simulink model "Sample_task"  (Simulink 8.1)
settings: Solver=ode4  SolverMode=SingleTasking  StartTime=0.0  StopTime=inf  FixedStep=0.0005  RelTol=1e-3
StartFcn:
  |  warndlg('Dexterit-E models cannot run under simulation. Please compile your model and run it from within Dexterit-E.');set_param(bdroot,'SimulationCommand','stop')
undefined symbols (not defined in the file or in its folder): slselsubs
libraries: simulink x4, General x3, KINARM_loads x2, KINARM_IO x1, KINARM_EP_loads x1, Video x1, xpclib x1
(part 2 of 3)

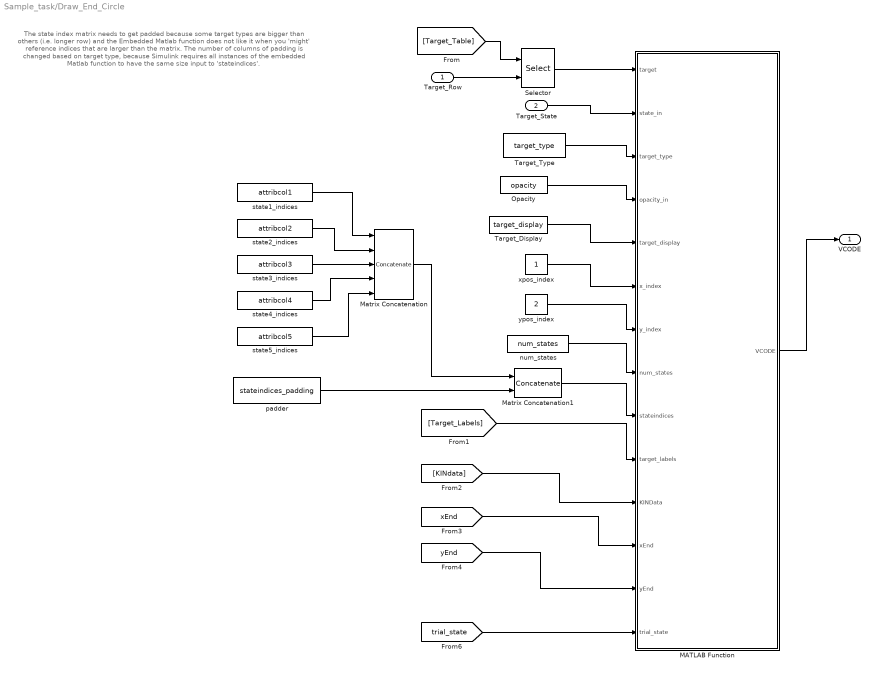
== system Sample_task/Draw_End_Circle ==
  note: The state index matrix needs to get padded because
      | some target types are bigger than others (i.e. longer row)
      | and the Embedded Matlab function does not like it when you
      |  'might' reference indices that are larger than the matrix.
      |
      | The number of columns of padding is changed based on target
      | type, because Simulink requires all instances of the embedded
      | Matlab function to have the same size input to 'stateindices'.
  Target_Row : Inport
  Target_State : Inport  Port=2
  MATLAB Function : MATLAB Function  TreatAsAtomicUnit=on
  Matrix Concatenation : Concatenate  NumInputs=5  Mode=Multidimensional array
  Matrix Concatenation1 : Concatenate  Mode=Multidimensional array  ConcatenateDimension=2
  Opacity : Constant  Value=opacity
  Selector : Selector  NumberOfDimensions=2  InputPortWidth=3  IndexOptions=Index vector (port),Select all  Indices=1,-1  OutputSizes=slselsubs([(-2),(-2)],1),slselsubs([(-2),(-2)],2)
  Target_Display : Constant  Value=target_display
  Target_Type : Constant  Value=target_type
  num_states : Constant  Value=num_states
  padder : Constant  Value=stateindices_padding
  state1_indices : Constant  Value=attribcol1  VectorParams1D=off
  state2_indices : Constant  Value=attribcol2  VectorParams1D=off
  state3_indices : Constant  Value=attribcol3  VectorParams1D=off
  state4_indices : Constant  Value=attribcol4  VectorParams1D=off
  state5_indices : Constant  Value=attribcol5  VectorParams1D=off
  xpos_index : Constant
  ypos_index : Constant  Value=2
  VCODE : Outport  PortDimensions=[1 70]
  wires:
  Target_Display/1 -> MATLAB Function/5(target_display)
  state2_indices/1 -> Matrix Concatenation/2
  state1_indices/1 -> Matrix Concatenation/1
  [Target_Labels] -> MATLAB Function/10(target_labels)
  Target_Row/1 -> Selector/2
  [Target_Table] -> Selector/1
  Selector/1 -> MATLAB Function/1(target)
  Target_State/1 -> MATLAB Function/2(state_in)
  MATLAB Function/1(VCODE) -> VCODE/1
  xpos_index/1 -> MATLAB Function/6(x_index)
  ypos_index/1 -> MATLAB Function/7(y_index)
  num_states/1 -> MATLAB Function/8(num_states)
  Matrix Concatenation/1 -> Matrix Concatenation1/1
  padder/1 -> Matrix Concatenation1/2
  Matrix Concatenation1/1 -> MATLAB Function/9(stateindices)
  state3_indices/1 -> Matrix Concatenation/3
  state4_indices/1 -> Matrix Concatenation/4
  state5_indices/1 -> Matrix Concatenation/5
  Opacity/1 -> MATLAB Function/4(opacity_in)
  Target_Type/1 -> MATLAB Function/3(target_type)
  [KINdata] -> MATLAB Function/11(KINData)
  [xEnd] -> MATLAB Function/12(xEnd)
  [yEnd] -> MATLAB Function/13(yEnd)
  [trial_state] -> MATLAB Function/14(trial_state)

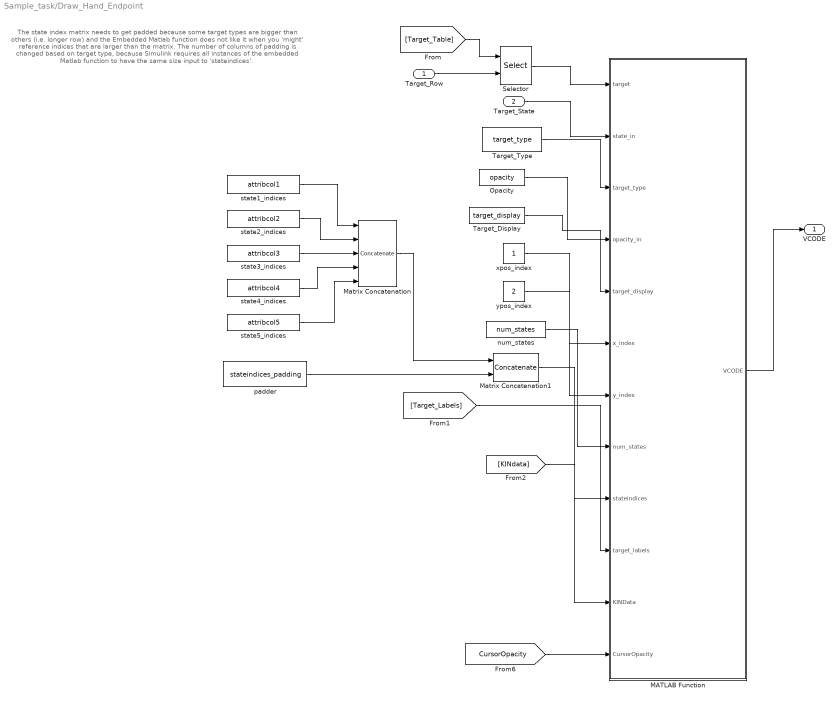
== system Sample_task/Draw_Hand_Endpoint ==
  note: The state index matrix needs to get padded because
      | some target types are bigger than others (i.e. longer row)
      | and the Embedded Matlab function does not like it when you
      |  'might' reference indices that are larger than the matrix.
      |
      | The number of columns of padding is changed based on target
      | type, because Simulink requires all instances of the embedded
      | Matlab function to have the same size input to 'stateindices'.
  Target_Row : Inport
  Target_State : Inport  Port=2
  MATLAB Function : MATLAB Function  TreatAsAtomicUnit=on
  Matrix Concatenation : Concatenate  NumInputs=5  Mode=Multidimensional array
  Matrix Concatenation1 : Concatenate  Mode=Multidimensional array  ConcatenateDimension=2
  Opacity : Constant  Value=opacity
  Selector : Selector  NumberOfDimensions=2  InputPortWidth=3  IndexOptions=Index vector (port),Select all  Indices=1,-1  OutputSizes=slselsubs([(-2),(-2)],1),slselsubs([(-2),(-2)],2)
  Target_Display : Constant  Value=target_display
  Target_Type : Constant  Value=target_type
  num_states : Constant  Value=num_states
  padder : Constant  Value=stateindices_padding
  state1_indices : Constant  Value=attribcol1  VectorParams1D=off
  state2_indices : Constant  Value=attribcol2  VectorParams1D=off
  state3_indices : Constant  Value=attribcol3  VectorParams1D=off
  state4_indices : Constant  Value=attribcol4  VectorParams1D=off
  state5_indices : Constant  Value=attribcol5  VectorParams1D=off
  xpos_index : Constant
  ypos_index : Constant  Value=2
  VCODE : Outport  PortDimensions=[1 70]
  wires:
  Target_Display/1 -> MATLAB Function/5(target_display)
  state2_indices/1 -> Matrix Concatenation/2
  state1_indices/1 -> Matrix Concatenation/1
  [Target_Labels] -> MATLAB Function/10(target_labels)
  Target_Row/1 -> Selector/2
  [Target_Table] -> Selector/1
  Selector/1 -> MATLAB Function/1(target)
  Target_State/1 -> MATLAB Function/2(state_in)
  MATLAB Function/1(VCODE) -> VCODE/1
  xpos_index/1 -> MATLAB Function/6(x_index)
  ypos_index/1 -> MATLAB Function/7(y_index)
  num_states/1 -> MATLAB Function/8(num_states)
  Matrix Concatenation/1 -> Matrix Concatenation1/1
  padder/1 -> Matrix Concatenation1/2
  Matrix Concatenation1/1 -> MATLAB Function/9(stateindices)
  state3_indices/1 -> Matrix Concatenation/3
  state4_indices/1 -> Matrix Concatenation/4
  state5_indices/1 -> Matrix Concatenation/5
  Opacity/1 -> MATLAB Function/4(opacity_in)
  Target_Type/1 -> MATLAB Function/3(target_type)
  [KINdata] -> MATLAB Function/11(KINData)
  [CursorOpacity] -> MATLAB Function/12(CursorOpacity)

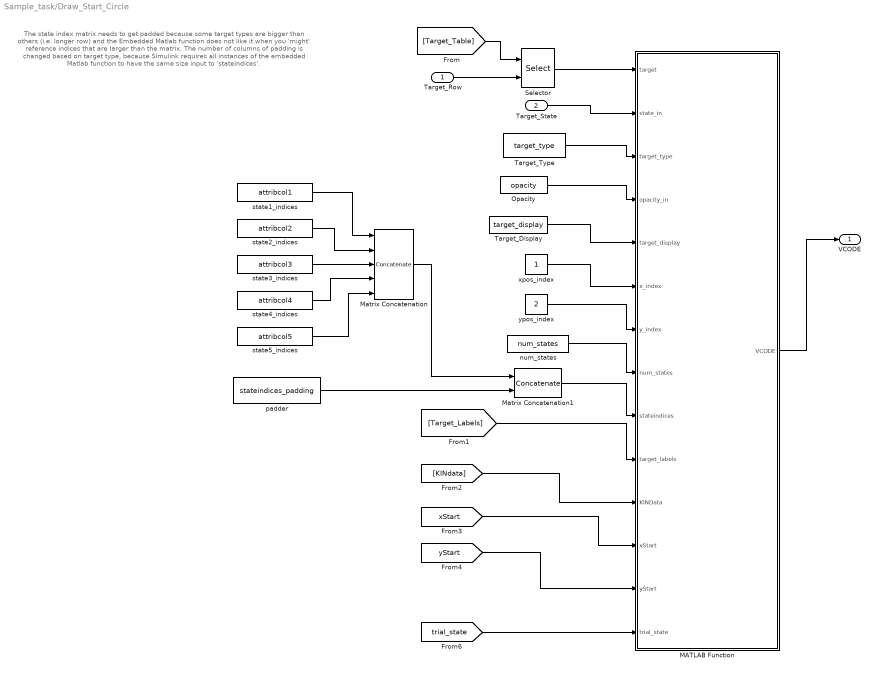
== system Sample_task/Draw_Start_Circle ==
  note: The state index matrix needs to get padded because
      | some target types are bigger than others (i.e. longer row)
      | and the Embedded Matlab function does not like it when you
      |  'might' reference indices that are larger than the matrix.
      |
      | The number of columns of padding is changed based on target
      | type, because Simulink requires all instances of the embedded
      | Matlab function to have the same size input to 'stateindices'.
  Target_Row : Inport
  Target_State : Inport  Port=2
  MATLAB Function : MATLAB Function  TreatAsAtomicUnit=on
  Matrix Concatenation : Concatenate  NumInputs=5  Mode=Multidimensional array
  Matrix Concatenation1 : Concatenate  Mode=Multidimensional array  ConcatenateDimension=2
  Opacity : Constant  Value=opacity
  Selector : Selector  NumberOfDimensions=2  InputPortWidth=3  IndexOptions=Index vector (port),Select all  Indices=1,-1  OutputSizes=slselsubs([(-2),(-2)],1),slselsubs([(-2),(-2)],2)
  Target_Display : Constant  Value=target_display
  Target_Type : Constant  Value=target_type
  num_states : Constant  Value=num_states
  padder : Constant  Value=stateindices_padding
  state1_indices : Constant  Value=attribcol1  VectorParams1D=off
  state2_indices : Constant  Value=attribcol2  VectorParams1D=off
  state3_indices : Constant  Value=attribcol3  VectorParams1D=off
  state4_indices : Constant  Value=attribcol4  VectorParams1D=off
  state5_indices : Constant  Value=attribcol5  VectorParams1D=off
  xpos_index : Constant
  ypos_index : Constant  Value=2
  VCODE : Outport  PortDimensions=[1 70]
  wires:
  Target_Display/1 -> MATLAB Function/5(target_display)
  state2_indices/1 -> Matrix Concatenation/2
  state1_indices/1 -> Matrix Concatenation/1
  [Target_Labels] -> MATLAB Function/10(target_labels)
  Target_Row/1 -> Selector/2
  [Target_Table] -> Selector/1
  Selector/1 -> MATLAB Function/1(target)
  Target_State/1 -> MATLAB Function/2(state_in)
  MATLAB Function/1(VCODE) -> VCODE/1
  xpos_index/1 -> MATLAB Function/6(x_index)
  ypos_index/1 -> MATLAB Function/7(y_index)
  num_states/1 -> MATLAB Function/8(num_states)
  Matrix Concatenation/1 -> Matrix Concatenation1/1
  padder/1 -> Matrix Concatenation1/2
  Matrix Concatenation1/1 -> MATLAB Function/9(stateindices)
  state3_indices/1 -> Matrix Concatenation/3
  state4_indices/1 -> Matrix Concatenation/4
  state5_indices/1 -> Matrix Concatenation/5
  Opacity/1 -> MATLAB Function/4(opacity_in)
  Target_Type/1 -> MATLAB Function/3(target_type)
  [KINdata] -> MATLAB Function/11(KINData)
  [xStart] -> MATLAB Function/12(xStart)
  [yStart] -> MATLAB Function/13(yStart)
  [trial_state] -> MATLAB Function/14(trial_state)

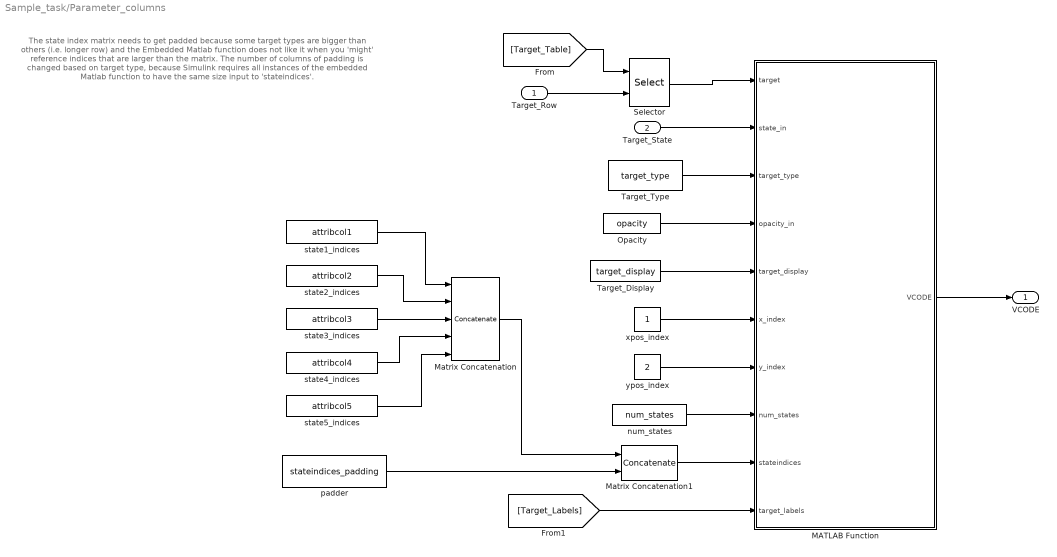
== system Sample_task/Parameter_columns ==
  note: The state index matrix needs to get padded because
      | some target types are bigger than others (i.e. longer row)
      | and the Embedded Matlab function does not like it when you
      |  'might' reference indices that are larger than the matrix.
      |
      | The number of columns of padding is changed based on target
      | type, because Simulink requires all instances of the embedded
      | Matlab function to have the same size input to 'stateindices'.
  Target_Row : Inport
  Target_State : Inport  Port=2
  MATLAB Function : MATLAB Function  TreatAsAtomicUnit=on
  Matrix Concatenation : Concatenate  NumInputs=5  Mode=Multidimensional array
  Matrix Concatenation1 : Concatenate  Mode=Multidimensional array  ConcatenateDimension=2
  Opacity : Constant  Value=opacity
  Selector : Selector  NumberOfDimensions=2  InputPortWidth=3  IndexOptions=Index vector (port),Select all  Indices=1,-1  OutputSizes=slselsubs([(-2),(-2)],1),slselsubs([(-2),(-2)],2)
  Target_Display : Constant  Value=target_display
  Target_Type : Constant  Value=target_type
  num_states : Constant  Value=num_states
  padder : Constant  Value=stateindices_padding
  state1_indices : Constant  Value=attribcol1  VectorParams1D=off
  state2_indices : Constant  Value=attribcol2  VectorParams1D=off
  state3_indices : Constant  Value=attribcol3  VectorParams1D=off
  state4_indices : Constant  Value=attribcol4  VectorParams1D=off
  state5_indices : Constant  Value=attribcol5  VectorParams1D=off
  xpos_index : Constant
  ypos_index : Constant  Value=2
  VCODE : Outport  PortDimensions=[1 70]
  wires:
  Target_Display/1 -> MATLAB Function/5(target_display)
  state2_indices/1 -> Matrix Concatenation/2
  state1_indices/1 -> Matrix Concatenation/1
  [Target_Labels] -> MATLAB Function/10(target_labels)
  Target_Row/1 -> Selector/2
  [Target_Table] -> Selector/1
  Selector/1 -> MATLAB Function/1(target)
  Target_State/1 -> MATLAB Function/2(state_in)
  MATLAB Function/1(VCODE) -> VCODE/1
  xpos_index/1 -> MATLAB Function/6(x_index)
  ypos_index/1 -> MATLAB Function/7(y_index)
  num_states/1 -> MATLAB Function/8(num_states)
  Matrix Concatenation/1 -> Matrix Concatenation1/1
  padder/1 -> Matrix Concatenation1/2
  Matrix Concatenation1/1 -> MATLAB Function/9(stateindices)
  state3_indices/1 -> Matrix Concatenation/3
  state4_indices/1 -> Matrix Concatenation/4
  state5_indices/1 -> Matrix Concatenation/5
  Opacity/1 -> MATLAB Function/4(opacity_in)
  Target_Type/1 -> MATLAB Function/3(target_type)

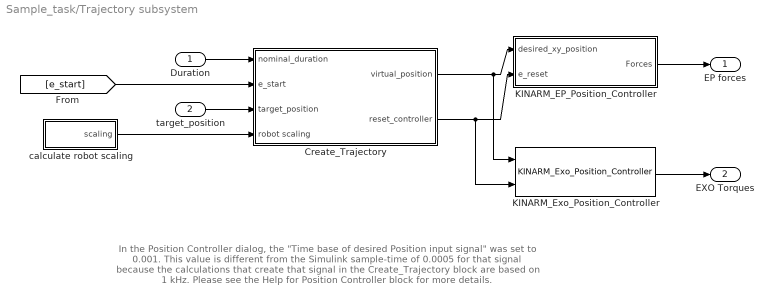
== system Sample_task/Trajectory subsystem ==
  note: In the Position Controller dialog, the "Time base of desired Position input signal" was set to 0.001.
      | This value is different from the Simulink sample-time of 0.0005 for that signal because the calculations
      | that create that signal in the Create_Trajectory block are based on 1 kHz. Please see the Help for
      | Position Controller block for more details.
  Duration : Inport
  target_position : Inport  Port=2
  Create_Trajectory : Subsystem
  KINARM_EP_Position_Controller : Subsystem  AncestorBlock=KINARM_EP_loads/KINARM_EP_Position_Controller  mask(KINARM_EP_Position_Controller){use_dom_hand=on, inertias_for_FF=KINARM End Point robot, gain_choice=Standard Movement, sample_time=0.001}
      mask prompts: use_dom_hand "Position control on dominant arm"; inertias_for_FF "Inertias to include for feed-forward control:"; gain_choice "Controller Performance"; sample_time "Time base of desired position input signal (-1 for inherited):"
      mask help:
      | <P>The KINARM_EP_Position_Controller block creates loads on the KINARM End-Point robot that implement position control of the hand using a feedforward model and feedback control.
      | <P>
      | The optional feedforward model uses estimates of KINARM End-Point robot inertia to create an estimate of required forces. A PD feedback controller is added to ensure optimal control.  The "Standard Movement" controller performance setting is optimized for reaching movements.  The "Step Response" setting is optimized for fast movements.
      | <P>
      | Desired position input is the (x, y) end-point position (i.e. handle).
      | <P>
      | <b>NOTE: it is critical to set the timebase of the desired position input signal correctly. Failure to do so will lead to robot instability, possibly damaging the KINARM robot and/or leading to subject injury.</b>
      mask init:
      | block_path = gcb;  % store block path, as gcb may change with block operations
      | 
      | %%% Handle background colours if link status changes.  
      | checkBackgroundColour(block_path, 'KINARM_EP_loads');
      | 
      | % Handle the inertias_for_FF setting: swap the 'inertia_option' inport with a constant block or 
      | % vice versa, if necessary, so that it matches the setting.
      | block_type = get_param([block_path '/inertia_option'], 'BlockType');
      | 
      | if (inertias_for_FF == 1) && ~strcmp(block_type, 'Inport') || ...  % if a change is required...
      |    (inertias_for_FF > 1) && strcmp(block_type, 'Inport')
      |     
      |     % ...delete the existing block, ...
      |     pos = get_param([block_path '/inertia_option'], 'Position');
      |     delete_line(block_path, 'inertia_option/1', 'FF_FB_Position_Controller/7');
      |     delete_block([block_path '/inertia_option']);
      |     
      |     % ...add an Inport or a 0-value Constant in place of the previous block (according to
      |     % the new setting), update the signal width flag, and then...
      |     if (inertias_for_FF == 1) && ~strcmp(block_type, 'Inport')
      |         add_block('built-in/Inport', [block_path '/inertia_option']);
      |      else
      |         add_block('built-in/Constant', [block_path '/inertia_option']);
      |         set_param([block_path '/inertia_option'], 'Value', 'inertias_for_FF - 2');
      |     end
      |     
      |     % ...connect the new block.
      |     set_param([block_path '/inertia_option'], 'Position', pos);
      |     add_line(block_path, 'inertia_option/1', 'FF_FB_Position_Controller/7');
      | end
      | 
      | 
      | 
      | % Set the sample rate of the desired_position input port based on the 
      | % sample rate from the mask
      | inports = find_system(block_path, 'LookUnderMasks', 'all', 'FollowLinks', 'on', 'SearchDepth', 1, 'BlockType', 'Inport');
      | set_param(inports{1}, 'SampleTime', get_param(gcb, 'sample_time') );
      | 
      | % Ensure the inports appear in a fixed order, and for each inport found add
      | % to the list of drawing commands a command to label it.
      | for i = 1:length(inports)
      |     inport_name = char(get_param(inports(i), 'Name'));
      |     
      |     if strcmp(inport_name, 'inertia_option')
      |         port = '3';
      | 	elseif strcmp(inport_name, 'desired_position')
      |         port = '1';
      |  	else
      | 		port = '2';
      | 		% do nothing
      | 	end
      |     
      |     set_param([block_path '/' inport_name], 'Port', port);
      | end
      mask Help:
      | Used to create loads for position control at the hand (i.e. finger-tip).
      | 
      | <H2>Library </H2>
      | KINARM_EP_loads (sub-library of Dexterit-E)
      | 
      | 
      | <H2>Description </H2>
      | The KINARM_EP_Position_Controller block creates loads on the KINARM End-Point robot that implement position control of the hand using a feedforward model and feedback control.
      | 
      | The optional feedforward model uses estimates of KINARM End-Point robot inertia to create an estimate of required forces. A PD feedback controller is added to ensure optimal control.  The "Standard Movement" controller performance setting is optimized for reaching movements.  The "Step Response" setting is optimized for fast movements.
      | <P>
      | <B>desired_xy_position: </B> this vector input is the desired position (i.e. attractor point) that the position controller acts on.  It should either be a [1x2] vector input or a VCODE.
      | The expected coordinate system and units for this input are the global coordinate system and meters.
      | <P>
      | <B>e_reset: </B> this scalar input resets the velocity and acceleration to zero for the feed-forward portion of the position controller model when e_reset transitions from 0 to 1.  This input should be used whenever the desired_xy_position input is being reset to a different position.
      | <P>
      | <B>inertia_option: </B> this optional scalar input defines which inertias to include for the feed-forward model.  Valid values are defined below.
      | <P>
      | <B>Forces: </B> this vector output is in a global Cartesian coordinate space as per all other KINARM End-Point load blocks.  It must be wired to the KINARM_EP_Apply_Loads block to actually apply the loads to the KINARM End-Point Robot.  This output may be added to other Force outputs from other KINARM End-Point load blocks to create a composite load.
      | <P>
      | 
      | <H2>Parameters and Dialog Box</H2>
      | <P>
      | <B>Position control on dominant arm:</B> indicates whether or not this position control is applied to the dominant arm (checked box) or non-dominant arm (unchecked box).
      | <P>
      | <B>Inertias to include for feed-forward control: </B> <BR>
      | Choices are: <BR>
      | (port)<BR>
      | 0 - None <BR>
      | 1 - KINARM End-Point robot  <BR>
      | <P>
      | If the (port) option is chosen, then an inport will be created allowing dynamic control of the inertia options.
      | The value wired to the inport will be mapped to the inertial choise using the values specified here (i.e. appropriate values are from 0-1).
      | Otherwise the option chosen will determine which inertias are included for the feed-forward control.
      | <P>
      | <B>Controller Performance: </B> <BR>
      | Choices are: <BR>
      | 1 - Standard Movement <BR>
      | 2 - Step Response  <BR>
      | <P>
      | The "Standard Movement" option is optimized for movements similar to normal reaching movements and provides high stiffness, but is underdamped.
      | There can be large overshoot following high accelerations/decellerations.
      | <P>
      | The "Step Response" option is optimized to minimize overshoot to less than ~10% for step responses, but at the cost of a reduction in controller stiffness.
      | <P>
      | NOTE: choice of Controller Performance option does not affect systems with secondary encoders - they are optimized for both conditions, providing higher stiffness and reasonable damping.
      | The controller for systems with secondary encoders provides less than ~10% overshoot for step responses.
      | <P>
      | 
      | <B>Time base of desired position input signal (-1 for inherited from sample time):</B> <BR>
      | Defines the time base used to calculate velocity and acceleration from the desired position input signal (-1 will inherit the time base from the sample time of the desired position input signal).
      | It is critical that this time base is set correctly.
      | The time base MUST be set to the time base used to create the desired input signal, WHICH MAY NOT BE THE SAME as the sample time of the desired input signal.
      | <B>Failure to set this time base correctly will lead to robot instability, possibly damaging the KINARM robot and/or leading to subject injury. </B>
      | <BR>
      | <I>Note: to determine the sample time of a signal, first update the model, then either select View --> Sample Time Legend or press Cntl + J.</I>
      | <P>
      | For example, a Stateflow chart that creates a desired position signal will, by default, use the model's sample time (e.g. 0.0005 s).
      | However, that Stateflow chart may use a time base that can be any multiple of the sample time (e.g. 0.001 s, 0.005 s, etc).
      | If a Stateflow chart was updating the desired position every 0.001 seconds, but the output sample time was 0.0005, then the position signal over time will look like:
      | <P>
      | [... x0, x0, x1, x1, x2, x2, x3, x3 ...].
      | <P>
      | A velocity calculated using 0.0005 time base will be:
      | <P>
      | [... 0, x1-x0, 0, x2-x1, 0, x3-x2, 0 ...] / 0.0005
      | <P>
      | (i.e. velocity will be 0 every other sample).
      | Whereas the true velocity in this example should be calculated using a 0.001 time base to create:
      | <P>
      |  [... x1-x0, x2-x1, x3-x2, ...] / 0.001.
      | 
      | <H2>Related Blocks </H2>
      | KINARM_EP_Apply_Loads, Virtual_Trajectory
      mask TypeOptions inertias_for_FF: (port) | None | KINARM End Point robot
      mask TypeOptions gain_choice: Standard Movement | Step Response
      mask Callback sample_time:
      | %ensure that sample time parameter is valid
      | sample_time_param = str2num( get_param(gcb, 'sample_time') );
      | model_step_size = str2num(get_param(bdroot, 'FixedStep'));
      | 
      | %default value:
      | sample_time = -1;
      | 
      | % if parameter value is numeric, sample_time_param will not be empty
      | if ~isempty(sample_time_param)
      | % 	round the sample time to an integer multiple of model step size, if possible
      | 	if ~isempty(model_step_size) && (model_step_size > 0)
      | 		sample_time = round( sample_time_param / model_step_size ) * model_step_size;
      | 	else
      | 		sample_time = sample_time_param;
      | 	end
      | 
      | 	% if input value is <=0, set it = -1 (inherited)
      | 	if (sample_time <= 0)
      | 		sample_time = -1;
      | 	end
      | end
      | 
      | set_param(gcb, 'sample_time', num2str(sample_time) );
  KINARM_Exo_Position_Controller : KINARM_loads/KINARM_Exo_Position_Controller  use_dom_hand=on  KINARM_Type=Human  inertias_for_FF=KINARM robot  angles_or_XY=End-point (global x/y)  sample_time=0.001
  calculate robot scaling : Subsystem
  EP forces : Outport
  EXO Torques : Outport  Port=2
  wires:
  Create_Trajectory/2(reset_controller) -> KINARM_EP_Position_Controller/2(e_reset), KINARM_Exo_Position_Controller/2
  Create_Trajectory/1(virtual_position) -> KINARM_EP_Position_Controller/1(desired_xy_position), KINARM_Exo_Position_Controller/1
  KINARM_EP_Position_Controller/1(Forces) -> EP forces/1
  KINARM_Exo_Position_Controller/1 -> EXO Torques/1
  target_position/1 -> Create_Trajectory/3(target_position)
  Duration/1 -> Create_Trajectory/1(nominal_duration)
  [e_start] -> Create_Trajectory/2(e_start)
  calculate robot scaling/1(scaling) -> Create_Trajectory/4(robot scaling)

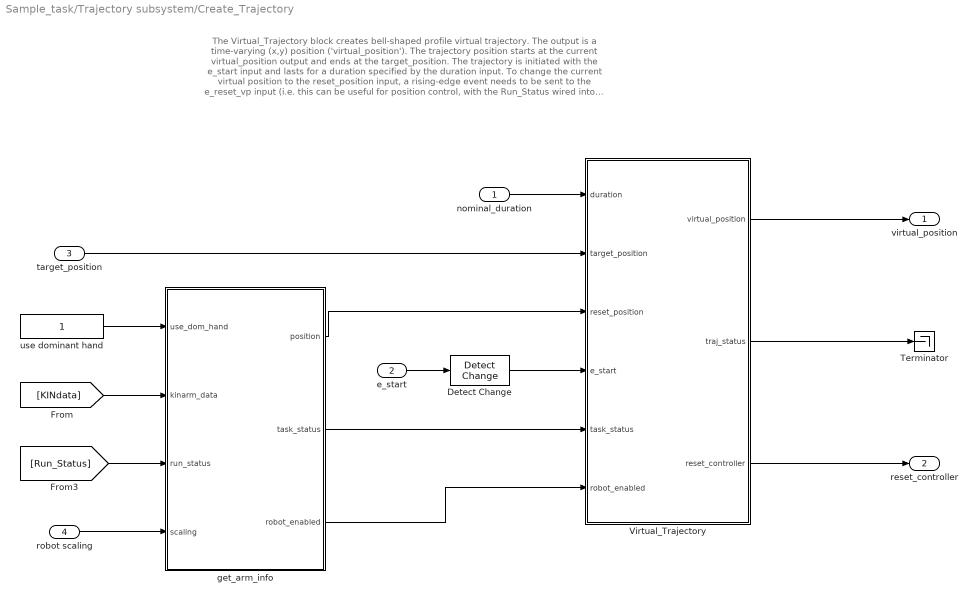
== system Sample_task/Trajectory subsystem/Create_Trajectory ==
  note: The Virtual_Trajectory block creates bell-shaped profile virtual trajectory.
      | The output is a time-varying (x,y) position ('virtual_position').
      |
      | The trajectory position starts at the current virtual_position output and ends at the target_position.
      | The trajectory is initiated with the e_start input and lasts for a duration specified by the duration input.
      |
      | To change the current virtual position to the reset_position input, a rising-edge event needs to be sent to the e_reset_vp input
      | (i.e. this can be useful for position control, with the Run_Status wired into the e_reset input).
      | If such an event occurs during a virtual trajectory, the trajectory is halted immediately.
  nominal_duration : Inport
  e_start : Inport  Port=2
  target_position : Inport  Port=3
  robot scaling : Inport  Port=4
  Detect Change : simulink/Logic and Bit Operations/Detect Change  vinit=0  InputProcessing=Inherited  OutDataTypeStr=uint8
  Terminator : Terminator
  Virtual_Trajectory : Subsystem
  get_arm_info : MATLAB Function  TreatAsAtomicUnit=on
  use dominant hand : Constant
  virtual_position : Outport
  reset_controller : Outport  Port=2
  wires:
  Virtual_Trajectory/1(virtual_position) -> virtual_position/1
  nominal_duration/1 -> Virtual_Trajectory/1(duration)
  e_start/1 -> Detect Change/1
  target_position/1 -> Virtual_Trajectory/2(target_position)
  Detect Change/1 -> Virtual_Trajectory/4(e_start)
  use dominant hand/1 -> get_arm_info/1(use_dom_hand)
  [KINdata] -> get_arm_info/2(kinarm_data)
  get_arm_info/1(position) -> Virtual_Trajectory/3(reset_position)
  Virtual_Trajectory/3(reset_controller) -> reset_controller/1
  get_arm_info/2(task_status) -> Virtual_Trajectory/5(task_status)
  get_arm_info/3(robot_enabled) -> Virtual_Trajectory/6(robot_enabled)
  [Run_Status] -> get_arm_info/3(run_status)
  Virtual_Trajectory/2(traj_status) -> Terminator/1
  robot scaling/1 -> get_arm_info/4(scaling)

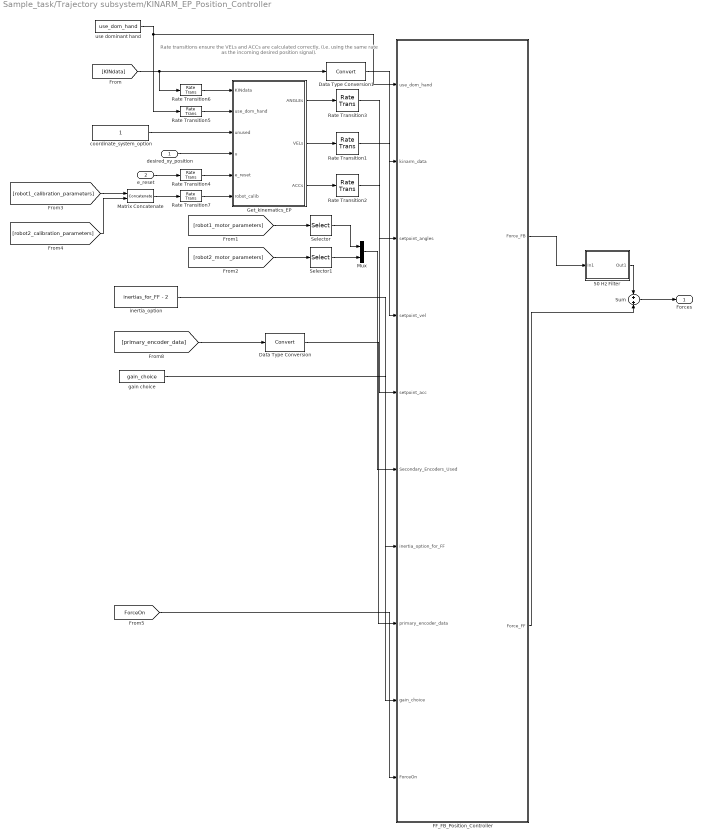
== system Sample_task/Trajectory subsystem/KINARM_EP_Position_Controller ==
  note: Rate transitions ensure the VELs and ACCs are calculated correctly,
      | (i.e. using the same rate as the incoming desired position signal).
  desired_xy_position : Inport  SampleTime=0.001
  e_reset : Inport  Port=2
  50 Hz Filter : Subsystem
  Data Type Conversion : DataTypeConversion
  Data Type Conversion1 : DataTypeConversion
  FF_FB_Position_Controller : MATLAB Function  TreatAsAtomicUnit=on
  Get_kinematics_EP : Subsystem  SystemSampleTime=.001
  Matrix Concatenate : Concatenate  Mode=Multidimensional array  ConcatenateDimension=2
  Mux : Mux  Inputs=2
  Rate Transition{1..7} (7 alike) : RateTransition
  Selector : Selector  IndexOptions=Index vector (dialog)  Indices=6  OutputSizes=[(-2)]
  Selector1 : Selector  IndexOptions=Index vector (dialog)  Indices=6  OutputSizes=[(-2)]
  Sum : Sum
  coordinate_system_option : Constant
  gain choice : Constant  Value=gain_choice
  inertia_option : Constant  Value=inertias_for_FF - 2
  use dominant hand : Constant  Value=use_dom_hand
  Forces : Outport  SampleTime=[0 1]
  wires:
  Data Type Conversion1/1 -> FF_FB_Position_Controller/2(kinarm_data)
  desired_xy_position/1 -> Get_kinematics_EP/4(u)
  use dominant hand/1 -> FF_FB_Position_Controller/1(use_dom_hand), Rate Transition5/1
  [KINdata] -> Data Type Conversion1/1, Rate Transition6/1
  Sum/1 -> Forces/1
  FF_FB_Position_Controller/1(Force_FB) -> 50 Hz Filter/1(In1)
  FF_FB_Position_Controller/2(Force_FF) -> Sum/2
  50 Hz Filter/1(Out1) -> Sum/1
  Get_kinematics_EP/1(ANGLEs) -> Rate Transition3/1
  Get_kinematics_EP/2(VELs) -> Rate Transition1/1
  Get_kinematics_EP/3(ACCs) -> Rate Transition2/1
  e_reset/1 -> Rate Transition4/1
  [robot1_motor_parameters] -> Selector/1
  [robot2_motor_parameters] -> Selector1/1
  Selector/1 -> Mux/1
  Selector1/1 -> Mux/2
  Mux/1 -> FF_FB_Position_Controller/6(Secondary_Encoders_Used)
  [primary_encoder_data] -> Data Type Conversion/1
  Data Type Conversion/1 -> FF_FB_Position_Controller/8(primary_encoder_data)
  gain choice/1 -> FF_FB_Position_Controller/9(gain_choice)
  Rate Transition1/1 -> FF_FB_Position_Controller/4(setpoint_vel)
  Rate Transition2/1 -> FF_FB_Position_Controller/5(setpoint_acc)
  Rate Transition3/1 -> FF_FB_Position_Controller/3(setpoint_angles)
  Rate Transition4/1 -> Get_kinematics_EP/5(e_reset)
  Rate Transition5/1 -> Get_kinematics_EP/2(use_dom_hand)
  Rate Transition6/1 -> Get_kinematics_EP/1(KINdata)
  coordinate_system_option/1 -> Get_kinematics_EP/3(unused)
  Rate Transition7/1 -> Get_kinematics_EP/6(robot_calib)
  Matrix Concatenate/1 -> Rate Transition7/1
  [robot1_calibration_parameters] -> Matrix Concatenate/1
  [robot2_calibration_parameters] -> Matrix Concatenate/2
  inertia_option/1 -> FF_FB_Position_Controller/7(inertia_option_for_FF)
  [ForceOn] -> FF_FB_Position_Controller/10(ForceOn)

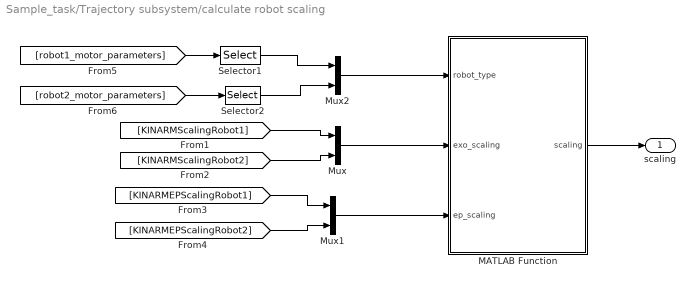
== system Sample_task/Trajectory subsystem/calculate robot scaling ==
  MATLAB Function : MATLAB Function  TreatAsAtomicUnit=on
  Mux : Mux  Inputs=2
  Mux1 : Mux  Inputs=2
  Mux2 : Mux  Inputs=2
  Selector1 : Selector  InputPortWidth=9  IndexOptions=Index vector (dialog)  Indices=[7]  OutputSizes=[(-2)]
  Selector2 : Selector  InputPortWidth=9  IndexOptions=Index vector (dialog)  Indices=[7]  OutputSizes=[(-2)]
  scaling : Outport
  wires:
  [KINARMScalingRobot1] -> Mux/1
  [KINARMScalingRobot2] -> Mux/2
  Mux/1 -> MATLAB Function/2(exo_scaling)
  Mux1/1 -> MATLAB Function/3(ep_scaling)
  Mux2/1 -> MATLAB Function/1(robot_type)
  MATLAB Function/1(scaling) -> scaling/1
  [robot2_motor_parameters] -> Selector2/1
  Selector2/1 -> Mux2/2
  [KINARMEPScalingRobot2] -> Mux1/2
  [KINARMEPScalingRobot1] -> Mux1/1
  Selector1/1 -> Mux2/1
  [robot1_motor_parameters] -> Selector1/1

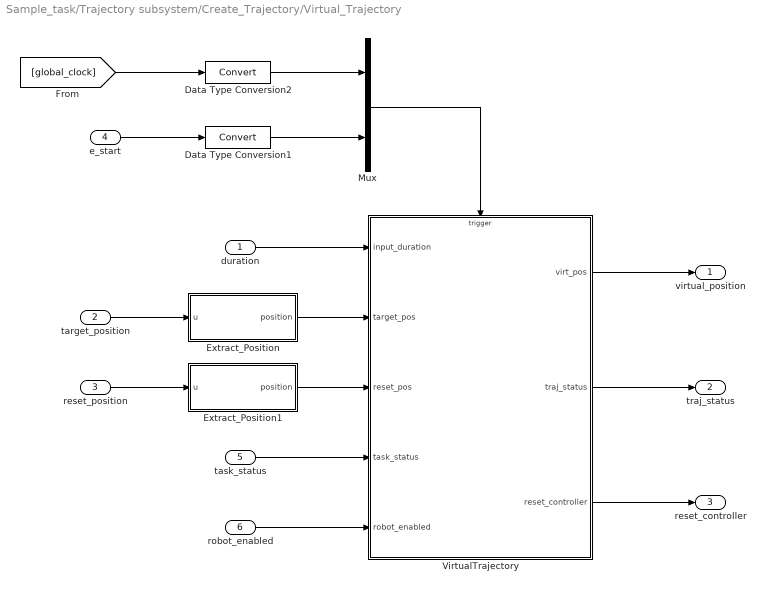
== system Sample_task/Trajectory subsystem/Create_Trajectory/Virtual_Trajectory ==
  duration : Inport
  target_position : Inport  Port=2
  reset_position : Inport  Port=3
  e_start : Inport  Port=4
  task_status : Inport  Port=5
  robot_enabled : Inport  Port=6
  Data Type Conversion1 : DataTypeConversion
  Data Type Conversion2 : DataTypeConversion
  Extract_Position : MATLAB Function  TreatAsAtomicUnit=on
  Extract_Position1 : MATLAB Function  TreatAsAtomicUnit=on
  Mux : Mux  Inputs=2
  VirtualTrajectory : Stateflow chart  TreatAsAtomicUnit=on
  virtual_position : Outport
  traj_status : Outport  Port=2
  reset_controller : Outport  Port=3
  wires:
  e_start/1 -> Data Type Conversion1/1
  target_position/1 -> Extract_Position/1(u)
  [global_clock] -> Data Type Conversion2/1
  Mux/1 -> VirtualTrajectory/Trigger
  duration/1 -> VirtualTrajectory/1(input_duration)
  VirtualTrajectory/1(virt_pos) -> virtual_position/1
  Extract_Position/1(position) -> VirtualTrajectory/2(target_pos)
  reset_position/1 -> Extract_Position1/1(u)
  Data Type Conversion2/1 -> Mux/1
  VirtualTrajectory/2(traj_status) -> traj_status/1
  robot_enabled/1 -> VirtualTrajectory/5(robot_enabled)
  task_status/1 -> VirtualTrajectory/4(task_status)
  Data Type Conversion1/1 -> Mux/2
  Extract_Position1/1(position) -> VirtualTrajectory/3(reset_pos)
  VirtualTrajectory/3(reset_controller) -> reset_controller/1

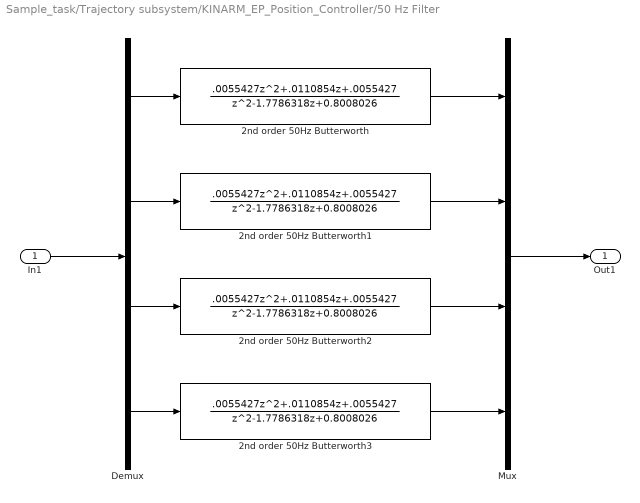
== system Sample_task/Trajectory subsystem/KINARM_EP_Position_Controller/50 Hz Filter ==
  In1 : Inport
  2nd order 50Hz Butterworth{,1..3} (4 alike) : DiscreteTransferFcn  Numerator=[.0055427 .0110854 .0055427]  Denominator=[1 -1.7786318 0.8008026]  SampleTime=.0005
  Demux : Demux
  Mux : Mux
  Out1 : Outport
  wires:
  Demux/2 -> 2nd order 50Hz Butterworth1/1
  In1/1 -> Demux/1
  Mux/1 -> Out1/1
  2nd order 50Hz Butterworth1/1 -> Mux/2
  Demux/1 -> 2nd order 50Hz Butterworth/1
  2nd order 50Hz Butterworth/1 -> Mux/1
  Demux/3 -> 2nd order 50Hz Butterworth2/1
  2nd order 50Hz Butterworth2/1 -> Mux/3
  Demux/4 -> 2nd order 50Hz Butterworth3/1
  2nd order 50Hz Butterworth3/1 -> Mux/4

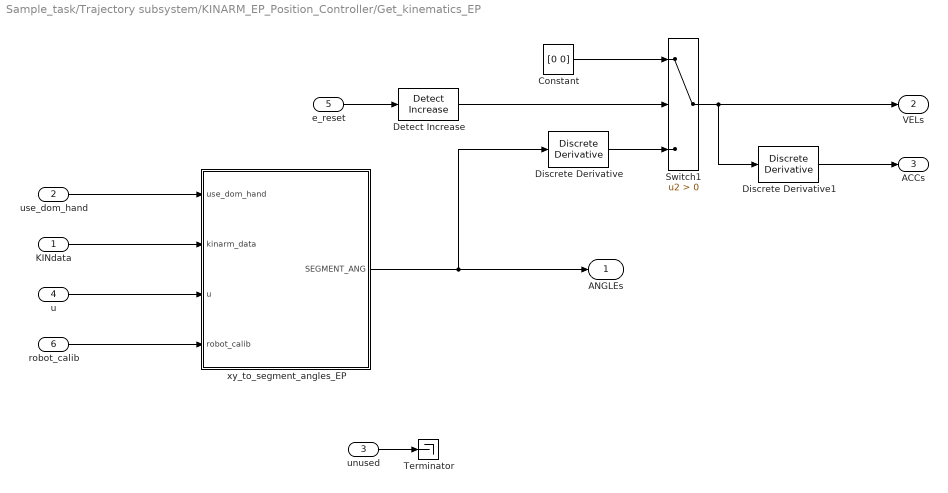
== system Sample_task/Trajectory subsystem/KINARM_EP_Position_Controller/Get_kinematics_EP ==
  KINdata : Inport
  use_dom_hand : Inport  Port=2
  unused : Inport  Port=3
  u : Inport  Port=4
  e_reset : Inport  Port=5
  robot_calib : Inport  Port=6
  Constant : Constant  Value=[0 0]
  Detect Increase : simulink/Logic and Bit Operations/Detect Increase  vinit=0.0  InputProcessing=Inherited  OutDataTypeStr=uint8
  Discrete Derivative : simulink/Discrete/Discrete Derivative  gainval=1.0  ICPrevScaledInput=0.0  InputProcessing=Inherited  OutMin=[]  OutMax=[]  OutDataType=sfix(16)  OutScaling=2^-10  DoSatur=off
  Discrete Derivative1 : simulink/Discrete/Discrete Derivative  gainval=1.0  ICPrevScaledInput=0.0  InputProcessing=Inherited  OutMin=[]  OutMax=[]  OutDataType=sfix(16)  OutScaling=2^-10  DoSatur=off
  Switch1 : Switch  Criteria=u2 > Threshold
  Terminator : Terminator
  xy_to_segment_angles_EP : MATLAB Function  TreatAsAtomicUnit=on
  ANGLEs : Outport
  VELs : Outport  Port=2
  ACCs : Outport  Port=3
  wires:
  xy_to_segment_angles_EP/1(SEGMENT_ANG) -> ANGLEs/1, Discrete Derivative/1
  Discrete Derivative/1 -> Switch1/3
  use_dom_hand/1 -> xy_to_segment_angles_EP/1(use_dom_hand)
  u/1 -> xy_to_segment_angles_EP/3(u)
  Switch1/1 -> Discrete Derivative1/1, VELs/1
  Constant/1 -> Switch1/1
  Detect Increase/1 -> Switch1/2
  Discrete Derivative1/1 -> ACCs/1
  KINdata/1 -> xy_to_segment_angles_EP/2(kinarm_data)
  e_reset/1 -> Detect Increase/1
  unused/1 -> Terminator/1
  robot_calib/1 -> xy_to_segment_angles_EP/4(robot_calib)

== stateflow chart Trial_Control ==
  settings: sampleTime=0.001
  state Main_Trial/
    state InCentre/
      rest = Trial_Protocol[REST_COL];
      % State - wait for subject
      trial_state = 0;
      % Initialize cursor
      EMG_trigger = 0;
    state EndOfTrial/
      logging_enable = 0;
      % State - rest
      trial_state = 2;
      EMG_trigger = 0;
    state DuringTrial/
      % Recording enabled
      logging_enable = 1;
      % Turn force on forever
      ForceOn = 1;
      % State - during trial
      trial_state = 1;
      % Trigger
      EMG_trigger = 5;
    state StayInCentre/
    StayInCentre -> InCentre [order 2] : [HandAtStart==0]
    InCentre -> StayInCentre : [HandAtStart==1]
    StayInCentre -> DuringTrial [order 1] : after(100,e_clk)
    DuringTrial -> EndOfTrial : after(Trial_Protocol[TRAJ_DURATION_COL]*1000,e_clk)
  state init/
    ForceOn = 0;
  state Inter_Trial_State/
    e_Trial_End
  state WaitForFlagToSet
  init -> InCentre
  (default) -> init
  Inter_Trial_State -> InCentre
  WaitForFlagToSet -> Inter_Trial_State : after(2, e_clk)
  Main_Trial -> WaitForFlagToSet : e_ExitTrialNow/
      | logging_enable = 0;
      | tickCount = 10;
  EndOfTrial -> Inter_Trial_State : after(rest*1000,e_clk)
  data: logging_enable output boolean; trial_state output double; tickCount local double; Trial_Protocol input double; HandAtStart input double; rest local double; ForceOn output double; EMG_trigger output double
  events: e_clk input RISING_EDGE_EVENT; e_ExitTrialNow input EITHER_EDGE_EVENT; e_Trial_End output EITHER_EDGE_EVENT

== matlab function Draw_End_Circle/MATLAB Function ==
  data: target input double; VCODE output double; state_in input double; target_type input double; opacity_in input double; target_display input double; x_index input double; y_index input double; num_states input double; stateindices input double; target_labels input double; KINData input double; xEnd input double; yEnd input double; trial_state input double
function VCODE = fcn(target, state_in, target_type, opacity_in, target_display, x_index, y_index, num_states, stateindices, target_labels, KINData, xEnd, yEnd, trial_state)

% stateindices should follow this order (depending on target-type):
% 1: fill colour
% 2: stroke colour
% 3: stroke width
% 4: major radius / radius / start point (line)
% 5: minor radius / end point (line)
% 6: orientation angle



% VCODEs are length 70. All units in a VCODE should be SI, e.g. (m) and (rad). Elements in a VCODE are defined as follows:
%
% For all target types:
%  1: target type
%       1 - circle
%       2 - ellipse
%       3 - rectangle
%       4 - line
%       5 - triangle
%       11 - circle with label
%       12 - ellipse with label
%       13 - rectangle with label
%       14 - line with label
%       15 - triangle with label
%  2: target on/off status and target display (which display target will appear on)
%		0 - off
%		1 - on, appearing on both subject and operator displays
%       2 - on, appearing on subject display only
%       3 - on, appearing on operator display only
%  3: x position (m)
%  4: y position (m)
%  5: fill colour (RRGGBB) or texture index
%  6: stroke colour (RRGGBB) or texture index
%  7: stroke width
%  8: reserved for target background ID
%  9: opacity
%
% For circles:
%  10: radius (m)
%
% For ellipses:
%  10: major radius (m)
%  11: minor radius (m)
%  12: orientation of major axis (rad)
%
% For rectangles:
%  10: length (m)
%  11: height (m)
%  12: orientation (rad) (relative to x, y already shown)
%
% For lines:
%  10: endpoint x-axis coordinate relative to start point (m)
%  11: endpoint y-axis coordinate relative to start point (m)
%
% For triangles:
%  10: length (m)
%  11: height (m)
%  12: offset of peak from midpoint of length (m)
%  13: orientation (rad)
%
% For all labelled target types:
%  14: reserved
%  15-64: label characters (indexes in ISO 8859-1 character set)
%  65: label colour (0xRRGGBB), opacity is set by the vcode's opacity (9).
%  66: label height (m)
%  67: reserved
%  68: reserved
%  69: reserved
%  70: reserved

num_targets = size(target, 1);

% NOTE: we assume that the STATE and/or OPACITY inputs are vectors. 

% If the length of the input STATE is not the same as the number of targets then make STATE a column vector of the same length as 
% the TARGET input, using the first STATE (i.e. all targets get the same state)
if num_targets == length(state_in)
	state = reshape(state_in, num_targets, 1);
else
	state = state_in(1) * ones(num_targets, 1);
end


% If the length of the input OPACITY is not the same as the number of targets then make OPACITY a column vector of the same length as
% the TARGET input, using the first OPACITY (i.e. all targets get the same opacity)
if num_targets == length(opacity_in)
	opacity = reshape(opacity_in, num_targets, 1);
else
	opacity = opacity_in(1) * ones(num_targets, 1);
end


% Clamping the opacity to [0, 100].
opacity = min(opacity, 100);
opacity = max(opacity, 0);

VCODE = zeros(num_targets, 70);

% Set the target type. Targets with labels have type codes 10 greater than their unlabelled counterparts.
VCODE(:, 1) = target_type + 10;

% Set the hand position.
VCODE(:, 3) = xEnd;  % x position (m)
VCODE(:, 4) = yEnd;  % y position (m)

for ii = 1:num_targets
	% Set the target on/off state. If the state input is 0, the target is off. Users of the VCODE should respect this
	% as an indication that the rest of the VCODE will be uninitialized.
	if (state(ii) <= 0) || (state(ii) > num_states)
		VCODE(ii, 2) = 0;  % target is off
	else
		VCODE(ii, 2) = target_display;  % Default is that target is on; target displays as specified by block mask
	end

	fill_colour_col = stateindices(state(ii), 1);
	stroke_colour_col = stateindices(state(ii), 2);
	stroke_width_col = stateindices(state(ii), 3);
	
	% Set the fill colour. Fill colour currently comes from the GUI in RRRGGGBBB format.
	%{
    if fill_colour_col == 0
		VCODE(ii, 5) = -2^31;
	elseif target(fill_colour_col) < 0
		VCODE(ii, 5) = target(ii, fill_colour_col);
	else
		VCODE(ii, 5) = colourshift(target(ii, fill_colour_col));
    end
    %}
    VCODE(ii,5) = colourshift(1000000000);
	
	% Set the stroke colour. Stroke colour currently comes from the GUI in RRRGGGBBB format.
    if trial_state==1
        if stroke_colour_col == 0
            VCODE(ii, 6) = -2^31;
        elseif target(stroke_colour_col) < 0
            VCODE(ii, 6) = target(ii, stroke_colour_col);
        else
            VCODE(ii, 6) = colourshift( target(ii, stroke_colour_col) );
        end
    else
        % CIRCLE APPEARS ONLY DURING TASK
        VCODE(ii, 6) = colourshift(1000000000);
    end

	% Set the stroke width. if target table index for stroke width is zero, then the stroke width is undefined
	if stroke_width_col == 0
		VCODE(ii, 7) = 0;                   % if stroke width column is 0, then stroke width is 0
	elseif stroke_width_col < 0
		VCODE(ii, 7) = 0.001;               % if stroke width column is -ve, then a 1mm default is chosen
	else
		VCODE(ii, 7) = target(ii, stroke_width_col) * 0.01;  % if stroke width column is +ve, convert width from (cm) in target table to (m)
    end

	% Set the opacity value
	VCODE(ii, 9) = opacity(ii);

	% Set attributes specific to each target type. In the process, note the first state vector column used for label information.
	label_index = 1;

	% Set attributes specific to each target type.
	if target_type == 1

		% Handle circle target:
		radius_col = stateindices(state(ii), 4);
		VCODE(ii, 10)=target(ii, radius_col);  % radius (in m)
	    label_index = 5;

	elseif target_type == 2 || target_type == 3

	    % Handle ellipse or rectangle target:
		major_col = stateindices(state(ii), 4);
		minor_col = stateindices(state(ii), 5);
		orientation_col = stateindices(state(ii), 6);
		
		VCODE(ii, 10) = target(ii, major_col) * 0.01;  % major radius (convert from (cm) in target table to (m))
		VCODE(ii, 11) = target(ii, minor_col) * 0.01;  % minor radius (convert from (cm) in target table to (m))
		if orientation_col == 0
			VCODE(ii, 12) = 0;  % if orientation column is 0, set orientation to 0 rad
		else
			VCODE(ii, 12) = mod(target(ii, orientation_col), 360) * pi / 180.0;  % orientation (convert from (degrees) in target table to (rad))
		end
	    label_index = 7;
	
	elseif target_type == 4

		% Handle line target:
		%xendpoint_col = stateindices(state(ii), 4);
		%yendpoint_col = stateindices(state(ii), 5);
		VCODE(ii, 10) = 0;  % line endpoint in x axis, relative to start (m)
		VCODE(ii, 11) = stateindices(state(ii), 1);  % line endpoint in y axis, relative to start (taken from Target Table)
	    label_index = 6;

	elseif target_type == 5

		% Handle triangle target:
		length_col = stateindices(state(ii), 4);
		height_col = stateindices(state(ii), 5);
		offset_col = stateindices(state(ii), 6);
		orientation_col = stateindices(state(ii), 7);

		VCODE(ii, 10) = target(ii, length_col) * 0.01;  % length (convert from (cm) in target table to (m))

		% If the height column is set to 0 then the triangle is automatically made equilateral, with the base length used as length
		% for all sides. If the height column is non-zero, separate values for height and peak offset are taken from the target table.
		if height_col == 0
			VCODE(ii, 11) = sin(pi / 3.0) * VCODE(ii, 10);  % height for equilateral triangle
			VCODE(ii, 12) = 0;                          % peak offset for equilateral triangle
		else
			VCODE(ii, 11) = target(ii, height_col) * 0.01;  % height (convert from (cm) in target table to (m))
			VCODE(ii, 12) = target(ii, offset_col) * 0.01;  % peak offset (convert from (cm) in target table to (m))
		end

		if orientation_col == 0
			VCODE(ii, 13) = 0;  % if orientation column is 0, set orientation to 0 rad
		else
			VCODE(ii, 13) = mod(target(ii, orientation_col), 360) * pi / 180.0;  % orientation (convert from (degrees) in target table to (rad))
		end
	    label_index = 8;
		
	end
	
	% Copy the label characters to the VCODE.
	for jj = 1:50
		VCODE(ii, jj + 14) = target_labels( target( ii, stateindices(state(ii), label_index) ), jj );
	end

	% Set the label colour. Like other colours, label colour comes from the GUI in RRRGGGBBB format and is converted to a 32-bit
	% 0xRRGGBB value here. If the target column table index for the colour is 0, the label is transparent.
	if stateindices(state(ii), label_index + 1) == 0
		VCODE(ii, 65) = -2^31;
	elseif target( ii, stateindices(state(ii), label_index + 1) ) < 0
		VCODE(ii, 65) = target( ii, stateindices(state(ii), label_index + 1) );
	else
		VCODE(ii, 65) = colourshift( target( ii, stateindices(state(ii), label_index + 1) ) );
	end

	% Set the label height. Label height is converted from (cm) in the target table to (m).
	VCODE(ii, 66) = target( ii, stateindices(state, label_index + 2) ) * 0.01;


	
end

% The colourshift function converts an "RRRGGGBBB" colour value to RRGBB (as an uint32).
function RRGGBBAA = colourshift(RRRGGGBBB)

%this is "no fill"
if RRRGGGBBB == 1000000000
    RRGGBBAA = cast(16777216, 'uint32'); %hex 0x1000000
    return; 
end

blue = cast(mod(RRRGGGBBB, 1000), 'uint32');
green = cast(mod(RRRGGGBBB - blue, 1000000) / 1000, 'uint32');
red = cast((RRRGGGBBB - (green * 1000) - blue) / 1000000, 'uint32');

RRGGBBAA = bitshift(red, 16) + bitshift(green, 8) + blue;

== matlab function Trajectory subsystem/Create_Trajectory/Virtual_Trajectory/Extract_Position ==
  settings: fimath=|
      | fimath(...
      | 'RoundMode', 'floor',...
      | 'OverflowMode', 'wrap',...
      | 'ProductMode', 'KeepLSB', 'ProductWordLength', 32,...
      | 'SumMode', 'KeepLSB', 'SumWordLength', 32,...
      | 'CastBeforeSum', false)
  data: u input double; position output double
function position = fcn(u)

position=[0,0];	%initialization
if length(u)==2	%input is assumed to be (x,y) position, global coordinates, (m)		
	position=u;
else			%input is assumed to be a VCODE
	position(1)=u(3);
	position(2)=u(4);
end

== matlab function function ==
  data: CursorOpacity output double; trial_state input double; TrialTimeOut output double; OpacityGradient input double
function [CursorOpacity,TrialTimeOut] = calculate_stuff(trial_state,OpacityGradient)

dt = 0.0005;

persistent trial_state_record; persistent TrialTime;
if isempty(trial_state_record), trial_state_record=0; TrialTime=0; end

if trial_state~=1
    % Timer is zero besides during task
    TrialTime = 0;
end
if trial_state_record==0 && trial_state==1
    % Reset time after trial begins
    TrialTime = 0;
end

% Calculate opacity
CursorOpacity = max(0,100*(1-TrialTime/OpacityGradient));

% Increment timer
TrialTime = TrialTime+dt;

% Output variables
TrialTimeOut = TrialTime;

% Record variable
trial_state_record = trial_state;

== matlab function Trajectory subsystem/Create_Trajectory/Virtual_Trajectory/Extract_Position1 ==
  settings: fimath=|
      | fimath(...
      | 'RoundMode', 'floor',...
      | 'OverflowMode', 'wrap',...
      | 'ProductMode', 'KeepLSB', 'ProductWordLength', 32,...
      | 'SumMode', 'KeepLSB', 'SumWordLength', 32,...
      | 'CastBeforeSum', false)
  data: u input double; position output double
function position = fcn(u)

position=[0,0];	%initialization
if length(u)==2	%input is assumed to be (x,y) position, global coordinates, (m)		
	position=u;
else			%input is assumed to be a VCODE
	position(1)=u(3);
	position(2)=u(4);
end

== matlab function Trajectory subsystem/calculate robot scaling/MATLAB Function ==
  data: robot_type input double; scaling output double; exo_scaling input double; ep_scaling input double
function scaling = fcn(robot_type, exo_scaling, ep_scaling)
%#codegen

scaling = [0, 0];

%0 = EXO, 1 = EP, 2 = NHP
for n=1:2
    if robot_type(n) == 1
        scaling(n) = ep_scaling(n);
    else
        scaling(n) = exo_scaling(n);
    end
end

== stateflow chart Trajectory subsystem/Create_Trajectory/Virtual_Trajectory/VirtualTrajectory ==
  state main/
    state wait_for_trigger/
      reset_controller = 0;
    state on_ramp/
      entry: tick = 0;    // initialize the tick counter
      reset_controller = 0;
      final_pos = target_pos;   // set the final position of the trajectory
      start_pos = virt_pos;   // set the start position of the trajectory
      duration = input_duration;   // store the duration of the trajectory
      traj_status = 1;   // indicate an ongoing trajectory
      during:
      on e_clk: tick++;
      // the trajectory velocity will have a bell shaped profile
      trajectory_shape = tick/duration-sin(2*pi*tick/duration)/(2*pi);
      virt_pos[1] = start_pos[1] + (final_pos[1] - start_pos[1]) * trajectory_shape;
      virt_pos[2] = start_pos[2] + (final_pos[2] - start_pos[2]) * trajectory_shape;
    state wait_1_ms_b/
      // wait for controller
      // to be reset
    main -> wait_1_ms_b [order 1] : [(robot_enabled == 1) && (traj_status == -1)]/
        | traj_status = 1;
        | virt_pos = reset_pos;
        | reset_controller = 1;
        | // trajectory was halted and
        | //is now being re-started
    wait_for_trigger -> (junction 93) : e_start
    (junction 93) -> wait_for_trigger [order 2]
    wait_1_ms_b -> (junction 93) : after(1, e_clk)
    (junction 93) -> on_ramp [order 1] : [input_duration>0]
    on_ramp -> wait_for_trigger [order 2] : [robot_enabled == 0]/
        | traj_status = -1;
        | // robot disabled
    on_ramp -> wait_for_trigger [order 1] : after(duration, e_clk)/
        | traj_status = 0
        | // trajectory completed
  state Initialization/
    virt_pos = reset_pos;
    // this initialization ensures that the virtual position
    // starts off as something reasonable
    traj_status = 0;   // initialize trajectory status
  state task_not_running/
    // wait for task_status to change
    // keep updating virt_pos so that the feedback
    // controller output, which is filtered, does not become
    // huge, resulting in a 'bump' if we don't do this.
    traj_status = 0;
    reset_controller = 0;
    during:
    virt_pos = reset_pos;
  state wait_1_ms/
    // wait for controller
    // to be reset
  (default) -> Initialization
  Initialization -> wait_for_trigger
  wait_1_ms -> wait_for_trigger : after(1, e_clk)
  task_not_running -> wait_1_ms : [task_status > 0]/
      | reset_controller = 1;
      | // task is running again,
      | // so reset position controller
  main -> task_not_running [order 1] : [task_status == 0]/
      | // means that run_status == 0
      | // AND that torque scaling at
      | // end of task is finished
  data: input_duration input double; target_pos input double size=[1 2]; tick local double; duration local double; reset_pos input double size=[1 2]; task_status input double; pi constant double =3.14159265358979; trajectory_shape local double; virt_pos output double size=[1 2]; traj_status output double; robot_enabled input double; start_pos local double size=[1 2]; final_pos local double size=[1 2]; reset_controller output double
  events: e_clk input RISING_EDGE_EVENT; e_start input RISING_EDGE_EVENT
